simulink model "SimulationPPU_Simscape"  (R2026a)
settings: Solver=ode23t  StopTime=10  MaxStep=1e-6  RelTol=1e-4
InitFcn:
  | % Read the SETTINGS constants on the top level
  | ppu_mdl = bdroot; ppu_mws = get_param(ppu_mdl, 'ModelWorkspace');
  | ppu_Fsw = slResolve(get_param([ppu_mdl '/Switching frequency'], 'Value'), ppu_mdl);
  | ppu_Vb  = slResolve(get_param([ppu_mdl '/DC bus voltage'], 'Value'), ppu_mdl);
  | assignin(ppu_mws, 'V_bus', ppu_Vb);            % initial DC-link voltage
  | set_param(ppu_mdl, 'MaxStep', sprintf('%.6g', 1/(20*ppu_Fsw)));
  | clear ppu_mdl ppu_mws ppu_Fsw ppu_Vb
model workspace (MAT data in the model file):
  C_cer = 3.36e-06
  C_elec = 0.0033
  C_f = 0.00088
  C_film = 4.5e-05
  ESR_cer = 0.0008
  ESR_elec = 0.023
  ESR_f = 0.057
  ESR_film = 0.0011
  Ki_I = 0.7
  Kp = 50
  Kp_I = 0.008
  L_Rser = 0.001
  L_f = 5.3e-05
  L_load = 0.0059
  N_par = 4
  R_Vsrc = 0.1
  R_load = 0.5
  Rb = 0.012
  Rd = 0.0092
  Rds_eq = 0.00440383953356
  Rg_ext = 1
  Rgs = 10000
  Ron_diode = 0.003
  Rs = 0.0069
  T_log = 2e-06
  T_stop = 0.2
  V_bus = 400
  Vf_diode = 0.65
  Vgs_on = 17.99820018
  Vhigh = 18
  Vto = 4.8
  m_max = 1.15470053838
  tau_Imeas = 0.001
libraries: fl_lib x23, nesl_utility x19, ee_lib x6, slpidlib x1, simulink x1
(part 2 of 2)

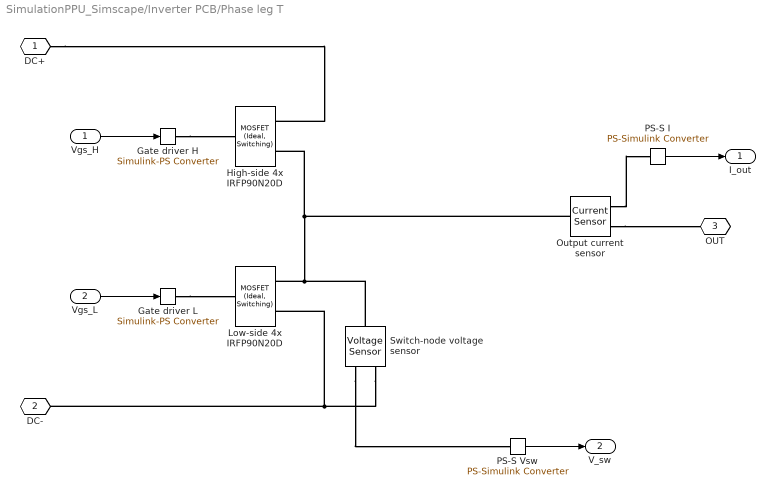
== system SimulationPPU_Simscape/Inverter PCB/Phase leg T ==
  Vgs_H : Inport
  Vgs_L : Inport  Port=2
  Gate driver H : nesl_utility/Simulink-PS Converter  PhysicalDomain=network_engine_domain  SubClassName=ps_input  LeftPortType=input  RightPortType=output  PseudoPeriodic=off  Frequencies=[]  NoiseDistribution=none  NoiseParameters=[]  Unit=V  AffineConversion=off  FilteringAndDerivatives=zero  SimscapeFilterOrder=1  InputFilterTimeConstant=0.001  UdotUserProvided=0
  Gate driver L : nesl_utility/Simulink-PS Converter  PhysicalDomain=network_engine_domain  SubClassName=ps_input  LeftPortType=input  RightPortType=output  PseudoPeriodic=off  Frequencies=[]  NoiseDistribution=none  NoiseParameters=[]  Unit=V  AffineConversion=off  FilteringAndDerivatives=zero  SimscapeFilterOrder=1  InputFilterTimeConstant=0.001  UdotUserProvided=0
  High-side 4x IRFP90N20D : ee_lib/Semiconductors & Converters/MOSFET (Ideal, Switching)  port_option=ee.enum.controlport.ps  Rds=Rds_eq Ohm  Goff=1e-7 1/Ohm  Vth=Vto V  diode_param=ee.enum.semiconductors.protectionDiode.nodynamics  diode_Vf=Vf_diode V  diode_Ron=Ron_diode Ohm  diode_Goff=1e-7 1/Ohm  diode_C=50e-9 F  diode_iRM=-235 A  diode_iF=300 A  diode_idot=-50 A/us  diode_trr_param=ee.enum.converters.diodeReverseParam.trr_factor  diode_trr_factor=3  diode_trr=15 us  diode_Qrr=1500 s*uA  ids_specify=off  ids_priority=None  ids=0 A  ids_nominal_specify=off  ids_nominal_value=1  ids_nominal_unit=A  vds_specify=off  vds_priority=None  vds=0 V  vds_nominal_specify=off  vds_nominal_value=1  vds_nominal_unit=V  vgs_specify=off  vgs_priority=None  vgs=0 V  vgs_nominal_specify=off  vgs_nominal_value=1  vgs_nominal_unit=V  thermal_loss_option=ee.enum.converters.thermalLossOption.constantvalues  Von_data=[0, 1.8, 3.2, 6, 10, 16; 0, 2, 5.5, 9.5, 15, 25] V  Tj=[298.15, 448.15] K  Iout_data=[0, 20, 40, 60, 80, 100] A  tabulateWithVds=false  Eon_data=[0, 55.04, 124.57, 235.53, 362.12; 0, 71.25, 161.25, 304.88, 468.75] * 1e-6 J  Eoff_data=[0, 18, 30, 56.1, 76.5; 0, 22.5, 37.5, 70.13, 95.63] * 1e-6 J  Eon_data_3D=[zeros(2, 5, 3)] J  Eoff_data_3D=[zeros(2, 5, 3)] J  Tj_loss=[298.15, 448.15] K  Iout_data_loss=[0, 10, 20, 30, 40] A  Vds_loss=[0, 150, 300] V  Eon_scalar=22.86e-3 J  Eoff_scalar=17.14e-3 J  Voff=300 V  Iout_scalar=600 A  useCurrentFromPreviousCycle=false  useVoltageFromPreviousCycle=false  diodeModelType=ee.enum.converters.diodeModelType.pwl  diodeTableType=ee.enum.diode.tableType.IfMat  diode_ReverseIVType=ee.enum.diode.diodeReverseIV.constant  diode_IfMat=[.07, .12, .19, 1.75, 4.24, 7.32, 11.2; .16, .3, .72, 2.14, 4.02, 6.35, 9.12] A  diode_VfMat=[.9, 1.15, 1.25, 1.5, 1.75, 2.17, 2.6, 2.85; .58, .68, .75, 1.1, 1.38, 1.77, 2.27, 2.7] V  diode_TjVec=[25, 125] degC  diode_VfVec=[.5, .7, .9, 1.3, 1.7, 2.1, 2.5] V  diode_IfVec=[.1, .2, .5, 1, 2, 4, 7, 10] A  diode_IrMat=[1e-06, 2e-06, 5e-06, 1e-05, 2.5e-05, 5e-05, .0001; 2e-06, 5e-06, 1e-05, 4e-05, 8e-05, .0002, .0005] A  diode_VrMat=[10, 100, 200, 250, 300, 325, 350; 10, 70, 160, 220, 270, 300, 320] V  diode_VrVec=[10, 20, 40, 50, 70, 80, 100] V  diode_IrVec=[1e-06, 2e-06, 5e-06, 1e-05, 2e-05, 5e-05, .0001] A  diode_Vr=-600 V  diode_Ls=150 nH  diode_Erec=0.03 J  diode_rec_loss_model=ee.enum.diode.reverseRecoveryModelTabulateUpTo3D.fixed  diode_ErecVal=0 J  diode_scaleWithIandV=true  diode_ErecMat=zeros(2, 3) J  diodeErecMat3D=zeros(2, 3, 2) J  diode_TjrecVec=[298.15, 398.15] K  diode_IfrecVec=[.1, 1, 10] A  diodeVrecVec=[0, 100] V  diode_IrecVal=10 A  diode_VrecVal=10 V  diode_tFilter=1 / 1000 / 100 s  separateThermalPortForDiode=false  thermal_network_parameterization=ee.enum.thermalNetworkTopology.external  Rth=[.03, .2] K/W  Rth_Cauer=[.03, .1, .2] K/W  Rth_Foster=[.08, .14, .22, .16] K/W  thermal_mass_parameterization=ee.enum.thermalNetwork.timeconstant  thermal_mass=[3, 25] J/K  thermal_mass_Cauer=[3, 10, 25] J/K  thermal_mass_Foster=[.001, .005, .05, .5] J/K  thermal_time_constant=[.1, 5] s  thermal_time_constant_Cauer=[.1, 1, 5] s  thermal_time_constant_Foster=[7e-05, .0007, .01, .08] s  thermal_mass_initial_temperatures=[25, 25] degC  thermal_mass_initial_temperatures_Cauer=[25, 25, 25] degC  junction_thermal_mass=0.1 J/K  Tvec_initial_Foster=[25, 25, 25, 25] degC  RthDiode=[.03, .2] K/W  RthCauerDiode=[.03, .1, .2] K/W  RthFosterDiode=[.03, .2] K/W  thermalMassDiode=[3, 25] J/K  thermalMassCauerDiode=[3, 10, 25] J/K  thermalMassFosterDiode=[33, 50] J/K  thermalTauDiode=[.1, 5] s  thermalTauCauerDiode=[.1, 1, 5] s  thermalTauFosterDiode=[1, 10] s  thermalMassInitTempDiode=[25, 25] degC  thermalMassInitTempCauerDiode=[25, 25, 25] degC  junctionthermalMassDiode=0.1 J/K  TVecInitialFosterDiode=[25, 25, 25, 25] degC  no_thermal_network=ee.enum.enable.no  mosfet_junction_temperature_specify=off  mosfet_junction_temperature_priority=None  mosfet_junction_temperature=25 degC  mosfet_junction_temperature_nominal_specify=off  mosfet_junction_temperature_nominal_value=1  mosfet_junction_temperature_nominal_unit=degC  diode_junction_temperature_specify=off  diode_junction_temperature_priority=None  diode_junction_temperature=25 degC  diode_junction_temperature_nominal_specify=off  diode_junction_temperature_nominal_value=1  diode_junction_temperature_nominal_unit=degC  Qj_specify=off  Qj_priority=None  Qj=0 W  Qj_nominal_specify=off  Qj_nominal_value=1  Qj_nominal_unit=W  accumulatedSwitchingLosses_specify=off  accumulatedSwitchingLosses_priority=None  accumulatedSwitchingLosses=0 J
  Low-side 4x IRFP90N20D : ee_lib/Semiconductors & Converters/MOSFET (Ideal, Switching)  port_option=ee.enum.controlport.ps  Rds=Rds_eq Ohm  Goff=1e-7 1/Ohm  Vth=Vto V  diode_param=ee.enum.semiconductors.protectionDiode.nodynamics  diode_Vf=Vf_diode V  diode_Ron=Ron_diode Ohm  diode_Goff=1e-7 1/Ohm  diode_C=50e-9 F  diode_iRM=-235 A  diode_iF=300 A  diode_idot=-50 A/us  diode_trr_param=ee.enum.converters.diodeReverseParam.trr_factor  diode_trr_factor=3  diode_trr=15 us  diode_Qrr=1500 s*uA  ids_specify=off  ids_priority=None  ids=0 A  ids_nominal_specify=off  ids_nominal_value=1  ids_nominal_unit=A  vds_specify=off  vds_priority=None  vds=0 V  vds_nominal_specify=off  vds_nominal_value=1  vds_nominal_unit=V  vgs_specify=off  vgs_priority=None  vgs=0 V  vgs_nominal_specify=off  vgs_nominal_value=1  vgs_nominal_unit=V  thermal_loss_option=ee.enum.converters.thermalLossOption.constantvalues  Von_data=[0, 1.8, 3.2, 6, 10, 16; 0, 2, 5.5, 9.5, 15, 25] V  Tj=[298.15, 448.15] K  Iout_data=[0, 20, 40, 60, 80, 100] A  tabulateWithVds=false  Eon_data=[0, 55.04, 124.57, 235.53, 362.12; 0, 71.25, 161.25, 304.88, 468.75] * 1e-6 J  Eoff_data=[0, 18, 30, 56.1, 76.5; 0, 22.5, 37.5, 70.13, 95.63] * 1e-6 J  Eon_data_3D=[zeros(2, 5, 3)] J  Eoff_data_3D=[zeros(2, 5, 3)] J  Tj_loss=[298.15, 448.15] K  Iout_data_loss=[0, 10, 20, 30, 40] A  Vds_loss=[0, 150, 300] V  Eon_scalar=22.86e-3 J  Eoff_scalar=17.14e-3 J  Voff=300 V  Iout_scalar=600 A  useCurrentFromPreviousCycle=false  useVoltageFromPreviousCycle=false  diodeModelType=ee.enum.converters.diodeModelType.pwl  diodeTableType=ee.enum.diode.tableType.IfMat  diode_ReverseIVType=ee.enum.diode.diodeReverseIV.constant  diode_IfMat=[.07, .12, .19, 1.75, 4.24, 7.32, 11.2; .16, .3, .72, 2.14, 4.02, 6.35, 9.12] A  diode_VfMat=[.9, 1.15, 1.25, 1.5, 1.75, 2.17, 2.6, 2.85; .58, .68, .75, 1.1, 1.38, 1.77, 2.27, 2.7] V  diode_TjVec=[25, 125] degC  diode_VfVec=[.5, .7, .9, 1.3, 1.7, 2.1, 2.5] V  diode_IfVec=[.1, .2, .5, 1, 2, 4, 7, 10] A  diode_IrMat=[1e-06, 2e-06, 5e-06, 1e-05, 2.5e-05, 5e-05, .0001; 2e-06, 5e-06, 1e-05, 4e-05, 8e-05, .0002, .0005] A  diode_VrMat=[10, 100, 200, 250, 300, 325, 350; 10, 70, 160, 220, 270, 300, 320] V  diode_VrVec=[10, 20, 40, 50, 70, 80, 100] V  diode_IrVec=[1e-06, 2e-06, 5e-06, 1e-05, 2e-05, 5e-05, .0001] A  diode_Vr=-600 V  diode_Ls=150 nH  diode_Erec=0.03 J  diode_rec_loss_model=ee.enum.diode.reverseRecoveryModelTabulateUpTo3D.fixed  diode_ErecVal=0 J  diode_scaleWithIandV=true  diode_ErecMat=zeros(2, 3) J  diodeErecMat3D=zeros(2, 3, 2) J  diode_TjrecVec=[298.15, 398.15] K  diode_IfrecVec=[.1, 1, 10] A  diodeVrecVec=[0, 100] V  diode_IrecVal=10 A  diode_VrecVal=10 V  diode_tFilter=1 / 1000 / 100 s  separateThermalPortForDiode=false  thermal_network_parameterization=ee.enum.thermalNetworkTopology.external  Rth=[.03, .2] K/W  Rth_Cauer=[.03, .1, .2] K/W  Rth_Foster=[.08, .14, .22, .16] K/W  thermal_mass_parameterization=ee.enum.thermalNetwork.timeconstant  thermal_mass=[3, 25] J/K  thermal_mass_Cauer=[3, 10, 25] J/K  thermal_mass_Foster=[.001, .005, .05, .5] J/K  thermal_time_constant=[.1, 5] s  thermal_time_constant_Cauer=[.1, 1, 5] s  thermal_time_constant_Foster=[7e-05, .0007, .01, .08] s  thermal_mass_initial_temperatures=[25, 25] degC  thermal_mass_initial_temperatures_Cauer=[25, 25, 25] degC  junction_thermal_mass=0.1 J/K  Tvec_initial_Foster=[25, 25, 25, 25] degC  RthDiode=[.03, .2] K/W  RthCauerDiode=[.03, .1, .2] K/W  RthFosterDiode=[.03, .2] K/W  thermalMassDiode=[3, 25] J/K  thermalMassCauerDiode=[3, 10, 25] J/K  thermalMassFosterDiode=[33, 50] J/K  thermalTauDiode=[.1, 5] s  thermalTauCauerDiode=[.1, 1, 5] s  thermalTauFosterDiode=[1, 10] s  thermalMassInitTempDiode=[25, 25] degC  thermalMassInitTempCauerDiode=[25, 25, 25] degC  junctionthermalMassDiode=0.1 J/K  TVecInitialFosterDiode=[25, 25, 25, 25] degC  no_thermal_network=ee.enum.enable.no  mosfet_junction_temperature_specify=off  mosfet_junction_temperature_priority=None  mosfet_junction_temperature=25 degC  mosfet_junction_temperature_nominal_specify=off  mosfet_junction_temperature_nominal_value=1  mosfet_junction_temperature_nominal_unit=degC  diode_junction_temperature_specify=off  diode_junction_temperature_priority=None  diode_junction_temperature=25 degC  diode_junction_temperature_nominal_specify=off  diode_junction_temperature_nominal_value=1  diode_junction_temperature_nominal_unit=degC  Qj_specify=off  Qj_priority=None  Qj=0 W  Qj_nominal_specify=off  Qj_nominal_value=1  Qj_nominal_unit=W  accumulatedSwitchingLosses_specify=off  accumulatedSwitchingLosses_priority=None  accumulatedSwitchingLosses=0 J
  Output current sensor : fl_lib/Electrical/Electrical Sensors/Current Sensor
  PS-S I : nesl_utility/PS-Simulink Converter  PhysicalDomain=network_engine_domain  SubClassName=ps_output  LeftPortType=input  RightPortType=output  PseudoPeriodic=off  Frequencies=[]  VectorFormat=inherit  Unit=inherit  AffineConversion=off
  PS-S Vsw : nesl_utility/PS-Simulink Converter  PhysicalDomain=network_engine_domain  SubClassName=ps_output  LeftPortType=input  RightPortType=output  PseudoPeriodic=off  Frequencies=[]  VectorFormat=inherit  Unit=inherit  AffineConversion=off
  Switch-node voltage sensor : fl_lib/Electrical/Electrical Sensors/Voltage Sensor
  DC+ : PMIOPort  Side=Left
  DC- : PMIOPort  Port=2  Side=Left
  OUT : PMIOPort  Port=3  Side=Right
  I_out : Outport
  V_sw : Outport  Port=2
  wires:
  Vgs_H/1 -> Gate driver H/1
  Vgs_L/1 -> Gate driver L/1
  PS-S I/1 -> I_out/1
  PS-S Vsw/1 -> V_sw/1
  connections:
  Gate driver H/RConn1 -- High-side 4x IRFP90N20D/LConn1
  Gate driver L/RConn1 -- Low-side 4x IRFP90N20D/LConn1
  DC+/RConn1 -- High-side 4x IRFP90N20D/RConn1
  Output current sensor/LConn1 -- High-side 4x IRFP90N20D/RConn2 -- Low-side 4x IRFP90N20D/RConn1 -- Switch-node voltage sensor/LConn1
  DC-/RConn1 -- Switch-node voltage sensor/RConn2 -- Low-side 4x IRFP90N20D/RConn2
  Output current sensor/RConn2 -- OUT/RConn1
  Output current sensor/RConn1 -- PS-S I/LConn1
  Switch-node voltage sensor/RConn1 -- PS-S Vsw/LConn1

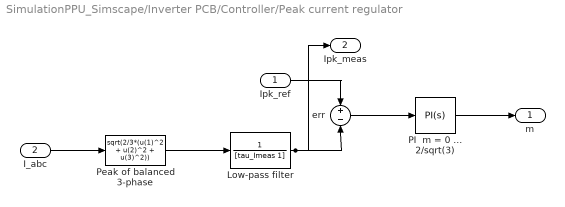
== system SimulationPPU_Simscape/Inverter PCB/Controller/Peak current regulator ==
  Ipk_ref : Inport
  I_abc : Inport  Port=2
  Low-pass filter : TransferFcn  Numerator=1  Denominator=[tau_Imeas 1]
  PI  m = 0 ... 2/sqrt(3) : slpidlib/PID Controller  Controller=PI  Form=Parallel  TimeDomain=Continuous-time  UseExternalTs=off  SampleTime=-1  IntegratorMethod=Forward Euler  FilterMethod=Forward Euler  ControllerParametersSource=internal  P=Kp_I  I=Ki_I  UseKiTs=off  D=0  UseExternalDerivativeSource=off  N=100  UseFilter=on  TunerSelectOption=Transfer Function Based (PID Tuner App)  ZeroCross=off  InitialConditionSource=internal  InitialConditionForIntegrator=0  InitialConditionForFilter=0  DifferentiatorICPrevScaledInput=0  ExternalReset=none  TrackingMode=off  Kt=1  LimitOutput=on  SatLimitsSource=internal  UpperSaturationLimit=m_max  LowerSaturationLimit=0  LinearizeAsGain=on  AntiWindupMode=clamping  Kb=1  LimitIntegrator=off  UpperIntegratorSaturationLimit=inf  LowerIntegratorSaturationLimit=-inf  POutMin=[]  POutMax=[]  IOutMin=[]  IOutMax=[]  DOutMin=[]  DOutMax=[]  NOutMin=[]  NOutMax=[]  SumOutMin=[]  SumOutMax=[]  SaturationOutMin=[]  SaturationOutMax=[]  PParamMin=[]  PParamMax=[]  IParamMin=[]  IParamMax=[]  DParamMin=[]  DParamMax=[]  NParamMin=[]  NParamMax=[]  KbParamMin=[]  KbParamMax=[]  KtParamMin=[]  KtParamMax=[]  KbOutMin=[]  KbOutMax=[]  KtOutMin=[]  KtOutMax=[]  IntegratorOutMin=[]  IntegratorOutMax=[]  FilterOutMin=[]  FilterOutMax=[]  SumI1OutMin=[]  SumI1OutMax=[]  SumI2OutMin=[]  SumI2OutMax=[]  SumI3OutMin=[]  SumI3OutMax=[]  SumI4OutMin=[]  SumI4OutMax=[]  SumDOutMin=[]  SumDOutMax=[]  DifferentiatorOutMin=[]  DifferentiatorOutMax=[]  FilterDiffOutCoefMin=[]  FilterDiffOutCoefMax=[]  ReciprocalOutMin=[]  ReciprocalOutMax=[]  SumDenOutMin=[]  SumDenOutMax=[]  SumNumOutMin=[]  SumNumOutMax=[]  DivideOutMin=[]  DivideOutMax=[]  UdiffTsProdOutMin=[]  UdiffTsProdOutMax=[]  NTsProdOutMin=[]  NTsProdOutMax=[]  UintegralTsProdOutMin=[]  UintegralTsProdOutMax=[]  UngainTsProdOutMin=[]  UngainTsProdOutMax=[]  ClampingZeroOutDataTypeStr=Inherit: Inherit via back propagation  ClampingZeroOutMin=[]  ClampingZeroOutMax=[]  FilterDenConstantOutDataTypeStr=Inherit: Inherit via back propagation  FilterDenConstantOutMin=[]  FilterDenConstantOutMax=[]  PCopyOutDataTypeStr=Inherit: Inherit via back propagation  PCopyOutMin=[]  PCopyOutMax=[]  NCopyOutDataTypeStr=Inherit: Inherit via back propagation  NCopyOutMin=[]  NCopyOutMax=[]  IntegratorContinuousStateAttributes=''  IntegratorStateMustResolveToSignalObject=off  IntegratorRTWStateStorageClass=Auto  FilterContinuousStateAttributes=''  FilterStateMustResolveToSignalObject=off  FilterRTWStateStorageClass=Auto  ParallelPVariant=InternalParameters  IdealPVariant=Disabled  IVariant=InternalParameters  DVariant=Disabled  IntegratorVariant=Continuous  SatVariant=Enabled  AWVariant=ContClampingParallel  PCopyVariant=Disabled  TRVariant=Disabled  FdbkBlocksVariant=Forward  IdealPFdbkVariant=Disabled  SatFdbkVariant=Disabled  DerivativeFilterVariant=Disabled  NVariant=Disabled  NCopyVariant=Disabled_SignalSpec  FilterICVariant=Disabled  IntegratorICVariant=InternalICs  ExternalResetVariant=Disabled  TRSumVariant=Passthrough  SumFdbkVariant=Disabled  SumVariant=Sum_PI  TsampFilterVariant=InternalTs  TsampNgainVariant=Passthrough  TsampIntegralVariant=Disabled_SignalSpec  ExternalSaturationOutDataTypeStr=Inherit: Same as second input  DerivativeSourceVariant=Disabled  PreIntVariant=InternalPreInt
  Peak of balanced 3-phase : Fcn  Expr=sqrt(2/3*(u(1)^2 + u(2)^2 + u(3)^2))
  err : Sum  Inputs=+-
  m : Outport
  Ipk_meas : Outport  Port=2
  wires:
  PI  m = 0 ... 2/sqrt(3)/1 -> m/1
  err/1 -> PI  m = 0 ... 2/sqrt(3)/1
  Low-pass filter/1 -> Ipk_meas/1, err/2
  Ipk_ref/1 -> err/1
  Peak of balanced 3-phase/1 -> Low-pass filter/1
  I_abc/1 -> Peak of balanced 3-phase/1

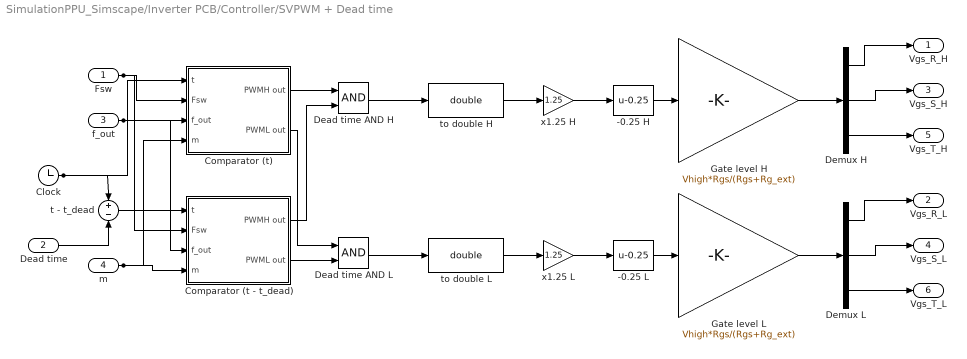
== system SimulationPPU_Simscape/Inverter PCB/Controller/SVPWM + Dead time ==
  Fsw : Inport
  Dead time : Inport  Port=2
  f_out : Inport  Port=3
  m : Inport  Port=4
  -0.25 H : Bias  Bias=-0.25  SaturateOnIntegerOverflow=off
  -0.25 L : Bias  Bias=-0.25  SaturateOnIntegerOverflow=off
  Clock : Clock
  Comparator (t - t_dead) : Subsystem
  Comparator (t) : Subsystem
  Dead time AND H : Logic  AllPortsSameDT=off  OutDataTypeStr=boolean
  Dead time AND L : Logic  AllPortsSameDT=off  OutDataTypeStr=boolean
  Demux H : Demux  Outputs=3
  Demux L : Demux  Outputs=3
  Gate level H : Gain  Gain=Vhigh*Rgs/(Rgs+Rg_ext)
  Gate level L : Gain  Gain=Vhigh*Rgs/(Rgs+Rg_ext)
  t - t_dead : Sum  Inputs=+-
  to double H : DataTypeConversion  OutDataTypeStr=double  SaturateOnIntegerOverflow=off  RndMeth=Floor
  to double L : DataTypeConversion  OutDataTypeStr=double  SaturateOnIntegerOverflow=off  RndMeth=Floor
  x1.25 H : Gain  Gain=1.25
  x1.25 L : Gain  Gain=1.25
  Vgs_R_H : Outport
  Vgs_R_L : Outport  Port=2
  Vgs_S_H : Outport  Port=3
  Vgs_S_L : Outport  Port=4
  Vgs_T_H : Outport  Port=5
  Vgs_T_L : Outport  Port=6
  wires:
  Demux L/3 -> Vgs_T_L/1
  Demux H/2 -> Vgs_S_H/1
  Demux H/1 -> Vgs_R_H/1
  Gate level L/1 -> Demux L/1
  -0.25 L/1 -> Gate level L/1
  -0.25 H/1 -> Gate level H/1
  to double L/1 -> x1.25 L/1
  x1.25 L/1 -> -0.25 L/1
  Clock/1 -> t - t_dead/1, Comparator (t)/1(t)
  to double H/1 -> x1.25 H/1
  Demux L/2 -> Vgs_S_L/1
  f_out/1 -> Comparator (t - t_dead)/3(f_out), Comparator (t)/3(f_out)
  Demux H/3 -> Vgs_T_H/1
  Dead time/1 -> t - t_dead/2
  Fsw/1 -> Comparator (t - t_dead)/2(Fsw), Comparator (t)/2(Fsw)
  Comparator (t - t_dead)/1(PWMH out) -> Dead time AND H/2
  t - t_dead/1 -> Comparator (t - t_dead)/1(t)
  Gate level H/1 -> Demux H/1
  Comparator (t - t_dead)/2(PWML out) -> Dead time AND L/2
  Demux L/1 -> Vgs_R_L/1
  x1.25 H/1 -> -0.25 H/1
  Comparator (t)/2(PWML out) -> Dead time AND L/1
  Dead time AND H/1 -> to double H/1
  Comparator (t)/1(PWMH out) -> Dead time AND H/1
  m/1 -> Comparator (t - t_dead)/4(m), Comparator (t)/4(m)
  Dead time AND L/1 -> to double L/1

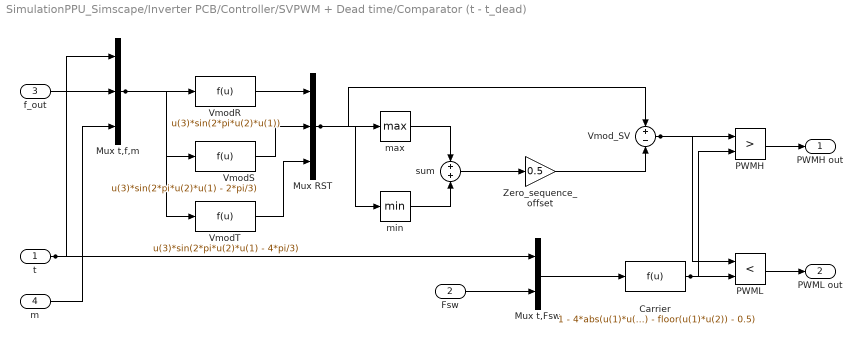
== system SimulationPPU_Simscape/Inverter PCB/Controller/SVPWM + Dead time/Comparator (t - t_dead) ==
  t : Inport
  Fsw : Inport  Port=2
  f_out : Inport  Port=3
  m : Inport  Port=4
  Carrier : Fcn  Expr=1 - 4*abs(u(1)*u(2) - floor(u(1)*u(2)) - 0.5)
  Mux RST : Mux  Inputs=3
  Mux t,Fsw : Mux  Inputs=2
  Mux t,f,m : Mux  Inputs=3
  PWMH : RelationalOperator  Operator=>  OutDataTypeStr=boolean  RndMeth=Simplest  InputSameDT=off
  PWML : RelationalOperator  Operator=<  OutDataTypeStr=boolean  RndMeth=Simplest  InputSameDT=off
  VmodR : Fcn  Expr=u(3)*sin(2*pi*u(2)*u(1))
  VmodS : Fcn  Expr=u(3)*sin(2*pi*u(2)*u(1) - 2*pi/3)
  VmodT : Fcn  Expr=u(3)*sin(2*pi*u(2)*u(1) - 4*pi/3)
  Vmod_SV : Sum  Inputs=+-
  Zero_sequence_offset : Gain  Gain=0.5
  max : MinMax  Function=max  ZeroCross=off
  min : MinMax  ZeroCross=off
  sum : Sum
  PWMH out : Outport
  PWML out : Outport  Port=2
  wires:
  Mux t,Fsw/1 -> Carrier/1
  f_out/1 -> Mux t,f,m/2
  PWML/1 -> PWML out/1
  m/1 -> Mux t,f,m/3
  PWMH/1 -> PWMH out/1
  Vmod_SV/1 -> PWML/1, PWMH/1
  t/1 -> Mux t,f,m/1, Mux t,Fsw/1
  Mux t,f,m/1 -> VmodT/1, VmodR/1, VmodS/1
  VmodR/1 -> Mux RST/1
  VmodT/1 -> Mux RST/3
  max/1 -> sum/1
  min/1 -> sum/2
  VmodS/1 -> Mux RST/2
  Mux RST/1 -> min/1, max/1, Vmod_SV/1
  sum/1 -> Zero_sequence_offset/1
  Fsw/1 -> Mux t,Fsw/2
  Carrier/1 -> PWML/2, PWMH/2
  Zero_sequence_offset/1 -> Vmod_SV/2

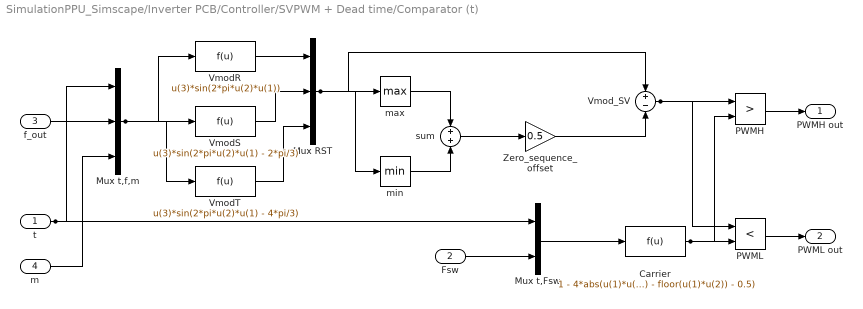
== system SimulationPPU_Simscape/Inverter PCB/Controller/SVPWM + Dead time/Comparator (t) ==
  t : Inport
  Fsw : Inport  Port=2
  f_out : Inport  Port=3
  m : Inport  Port=4
  Carrier : Fcn  Expr=1 - 4*abs(u(1)*u(2) - floor(u(1)*u(2)) - 0.5)
  Mux RST : Mux  Inputs=3
  Mux t,Fsw : Mux  Inputs=2
  Mux t,f,m : Mux  Inputs=3
  PWMH : RelationalOperator  Operator=>  OutDataTypeStr=boolean  RndMeth=Simplest  InputSameDT=off
  PWML : RelationalOperator  Operator=<  OutDataTypeStr=boolean  RndMeth=Simplest  InputSameDT=off
  VmodR : Fcn  Expr=u(3)*sin(2*pi*u(2)*u(1))
  VmodS : Fcn  Expr=u(3)*sin(2*pi*u(2)*u(1) - 2*pi/3)
  VmodT : Fcn  Expr=u(3)*sin(2*pi*u(2)*u(1) - 4*pi/3)
  Vmod_SV : Sum  Inputs=+-
  Zero_sequence_offset : Gain  Gain=0.5
  max : MinMax  Function=max  ZeroCross=off
  min : MinMax  ZeroCross=off
  sum : Sum
  PWMH out : Outport
  PWML out : Outport  Port=2
  wires:
  Carrier/1 -> PWML/2, PWMH/2
  Vmod_SV/1 -> PWML/1, PWMH/1
  Mux t,f,m/1 -> VmodT/1, VmodS/1, VmodR/1
  max/1 -> sum/1
  Mux t,Fsw/1 -> Carrier/1
  m/1 -> Mux t,f,m/3
  t/1 -> Mux t,f,m/1, Mux t,Fsw/1
  VmodR/1 -> Mux RST/1
  PWML/1 -> PWML out/1
  Fsw/1 -> Mux t,Fsw/2
  VmodS/1 -> Mux RST/2
  sum/1 -> Zero_sequence_offset/1
  PWMH/1 -> PWMH out/1
  VmodT/1 -> Mux RST/3
  Mux RST/1 -> min/1, max/1, Vmod_SV/1
  f_out/1 -> Mux t,f,m/2
  min/1 -> sum/2
  Zero_sequence_offset/1 -> Vmod_SV/2
